simulink model "control_pmsm_multiple_wrapped"  (R2024b)
settings: Solver=FixedStepAuto  StartTime=0.0  StopTime=1  RelTol=1e-3  EnableMultiTasking=on
undefined symbols (not defined in the file): ControlModes, EstimationVelocityModes, InitConfParams, SupervisorEvents
settings Model: DataDictionary=amcfoc.sldd  Creator=upattacini  LastModifiedBy=mfussi
settings SolverCC: AllowMultiTaskInputOutput=on  AutoInsertRateTranBlk=on  InsertRTBMode=Never (minimum delay)  EnableFixedStepZeroCrossing=on
settings DataIOCC: SaveOutput=off  SignalLogging=off  DSMLogging=off  SaveTime=off
settings OptimizationCC: UseDivisionForNetSlopeComputation=on  SimCompilerOptimization=on
settings DebuggingCC: ParameterPrecisionLossMsg=none  UnconnectedInputMsg=warning  UnconnectedOutputMsg=warning  UnconnectedLineMsg=warning  BusObjectLabelMismatch=none
settings ModelReferenceCC: EnableRefExpFcnMdlSchedulingChecks=on  ModelReferenceMinAlgLoopOccurrences=on
settings SFSimCC: SimHardwareAcceleration=native
settings RTWCC: Toolchain=MinGW64 | gmake (64-bit Windows)  BuildConfiguration=Faster Runs  GPUComputeCapability=3.5  DLArmComputeVersion=19.05
settings GRTTargetCC: CodeInterfacePackaging=Reusable function  GenerateAllocFcn=on

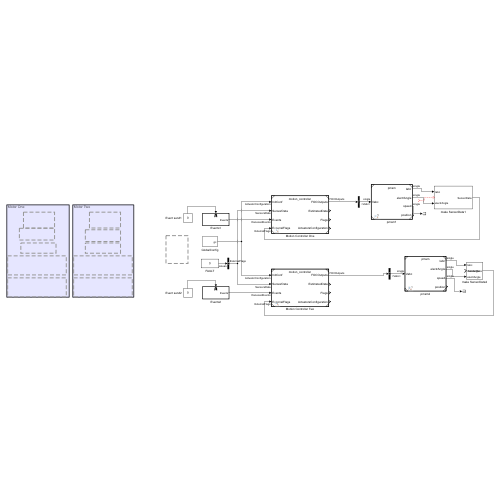
[thumbnail: Simulink's stored preview of the top-level diagram]
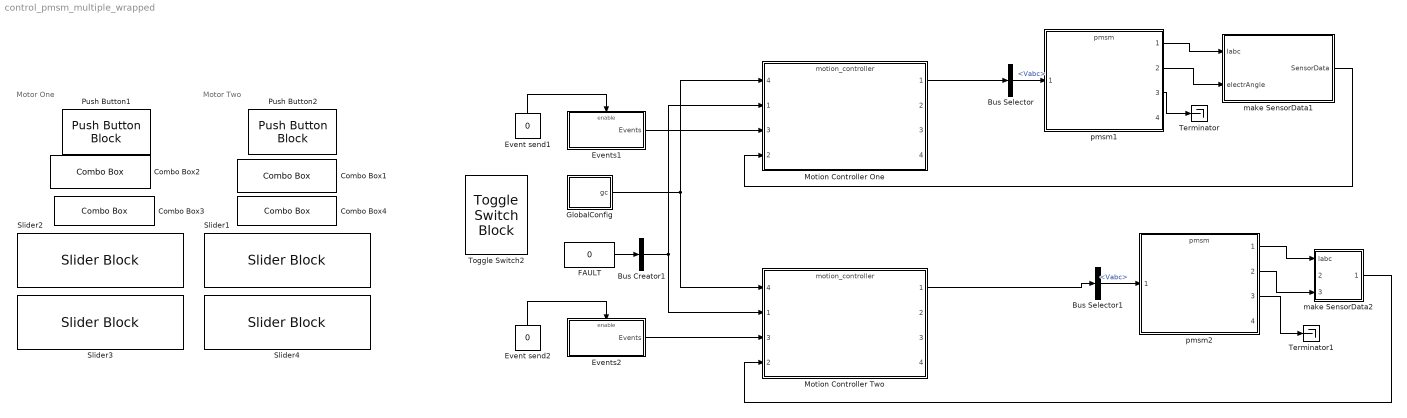
== system control_pmsm_multiple_wrapped ==
  note: Motor One
  note: Motor Two
  Bus Creator1 : BusCreator  Inputs=1  OutDataTypeStr=Bus: ExternalFlags  NonVirtualBus=on
      settings: InheritFromInputs=off
  Bus Selector : BusSelector  OutputSignals=Vabc
  Bus Selector1 : BusSelector  OutputSignals=Vabc
  Combo Box1 : ComboBox  SelectedLabel=None  UseEnumeratedDataType=on  EnumeratedDataType=SupervisorEvents
      settings: Values={{'None', 'SetLimit', 'SetControlMode', 'SetMotorConfig', 'SetPid', 'SetTarget'}, [0 1 2 5 3 4]}
  Combo Box2 : ComboBox  SelectedLabel=None  UseEnumeratedDataType=on  EnumeratedDataType=SupervisorEvents
      settings: Values={{'None', 'SetLimit', 'SetControlMode', 'SetMotorConfig', 'SetPid', 'SetTarget'}, [0 1 2 5 3 4]}
  Combo Box3 : ComboBox  SelectedLabel=Current  UseEnumeratedDataType=on  EnumeratedDataType=ControlModes
      settings: Values={{'NotConfigured', 'Idle', 'Position', 'PositionDirect', 'Current', 'Velocity', 'Voltage', 'Torque', 'HwFaultCM'}, [0 1 2 3 4 5 6 7 8]}
  Combo Box4 : ComboBox  SelectedLabel=Current  UseEnumeratedDataType=on  EnumeratedDataType=ControlModes
      settings: Values={{'NotConfigured', 'Idle', 'Position', 'PositionDirect', 'Current', 'Velocity', 'Voltage', 'Torque', 'HwFaultCM'}, [0 1 2 3 4 5 6 7 8]}
  Event send1 : Constant  Value=0
  Event send2 : Constant  Value=0
  Events1 : Subsystem
  Events2 : Subsystem
  FAULT : Constant  Value=0  OutDataTypeStr=Inherit: Inherit via back propagation
  GlobalConfig : Subsystem
  Motion Controller One : ModelReference  ModelNameDialog=motion_controller.slx  SimulationMode=Normal  ModelReferenceVersion=4.0
      settings: PortSchema="{\"entries\":[{\"content\":{\"sides\":[{\"content\":{\"connectorIds\":[\"In4\",\"In1\",\"In3\",\"In2\"]},\"type\":\"ConnectorPlacement.EquallySpacedRectSide\",\"uuid\":\"9501764e-0215-4e66-aa8b-5739ba26e582\"},{\"content\":{\"connectorIds\":[\"Out1\",\"Out2\",\"Out3\",\"Out4\"],\"side\":\"RIGHT\"},\"type\":\"ConnectorPlacement.EquallySpacedRectSide\",\"uuid\":\"34be47de-e9bc-43ca-97ac-58a43ba9eb9a\"},{\"content\":{\"side\":\"TOP\"},\"type\":\"ConnectorPlacement.EquallySpacedRectSide\",\"uuid\":\"71d421f6-ab26-4482-875c-bb9e44468ca7\"}]},\"type\":\"ConnectorPlacement.EquallySpacedConnector\",\"uuid\":\"be89792d-26da-4e9c-8783-03826ec72805\"}],\"packageUris\":[\"http://schema.mathworks.com/mf0/Connector/R2020b\"],\"version\":\"1.0\"}"
  Motion Controller Two : ModelReference  ModelNameDialog=motion_controller.slx  SimulationMode=Normal  ModelReferenceVersion=4.0
      settings: PortSchema="{\"entries\":[{\"content\":{\"sides\":[{\"content\":{\"connectorIds\":[\"In4\",\"In1\",\"In3\",\"In2\"]},\"type\":\"ConnectorPlacement.EquallySpacedRectSide\",\"uuid\":\"9501764e-0215-4e66-aa8b-5739ba26e582\"},{\"content\":{\"connectorIds\":[\"Out1\",\"Out2\",\"Out3\",\"Out4\"],\"side\":\"RIGHT\"},\"type\":\"ConnectorPlacement.EquallySpacedRectSide\",\"uuid\":\"34be47de-e9bc-43ca-97ac-58a43ba9eb9a\"},{\"content\":{\"side\":\"TOP\"},\"type\":\"ConnectorPlacement.EquallySpacedRectSide\",\"uuid\":\"71d421f6-ab26-4482-875c-bb9e44468ca7\"}]},\"type\":\"ConnectorPlacement.EquallySpacedConnector\",\"uuid\":\"be89792d-26da-4e9c-8783-03826ec72805\"}],\"packageUris\":[\"http://schema.mathworks.com/mf0/Connector/R2020b\"],\"version\":\"1.0\"}"
  Push Button1 : PushButtonBlock  LabelPosition=Top  OffValue=0.000000
  Push Button2 : PushButtonBlock  LabelPosition=Top  OffValue=0.000000
  Slider1 : SliderBlock  ScaleMax=1
  Slider2 : SliderBlock  ScaleMax=1
  Slider3 : SliderBlock  ScaleMax=0.36
  Slider4 : SliderBlock  ScaleMax=0.36
  Terminator : Terminator
  Terminator1 : Terminator
  Toggle Switch2 : ToggleSwitchBlock
      settings: Values={{'Off', 'On'}, [0 1]}
  make SensorData1 : Subsystem
  make SensorData2 : Subsystem
  pmsm1 : ModelReference  ModelNameDialog=pmsm.slx  SimulationMode=Normal  ModelReferenceVersion=9.5
  pmsm2 : ModelReference  ModelNameDialog=pmsm.slx  SimulationMode=Normal  ModelReferenceVersion=9.5
  wires:
  Event send1/1 -> Events1/Enable
  FAULT/1 -> Bus Creator1/1
  pmsm1/1 -> make SensorData1/1(Iabc)
  ? -> ?
  pmsm1/2 -> make SensorData1/2(electrAngle)
  pmsm2/1 -> make SensorData2/1(Iabc)
  pmsm2/2 -> make SensorData2/3(electrAngle)
  pmsm1/3 -> Terminator/1
  pmsm2/3 -> Terminator1/1
  Event send2/1 -> Events2/Enable
  Motion Controller One/1 -> Bus Selector/1
  Bus Selector/1 -> pmsm1/1  "<Vabc>"
  Motion Controller Two/1 -> Bus Selector1/1
  Bus Selector1/1 -> pmsm2/1  "<Vabc>"
  GlobalConfig/1(gc) -> Motion Controller One/4, Motion Controller Two/4
  Bus Creator1/1 -> Motion Controller One/1, Motion Controller Two/1
  Events1/1(Events) -> Motion Controller One/3
  make SensorData2/1(SensorData) -> Motion Controller Two/2
  Events2/1(Events) -> Motion Controller Two/3
  make SensorData1/1(SensorData) -> Motion Controller One/2

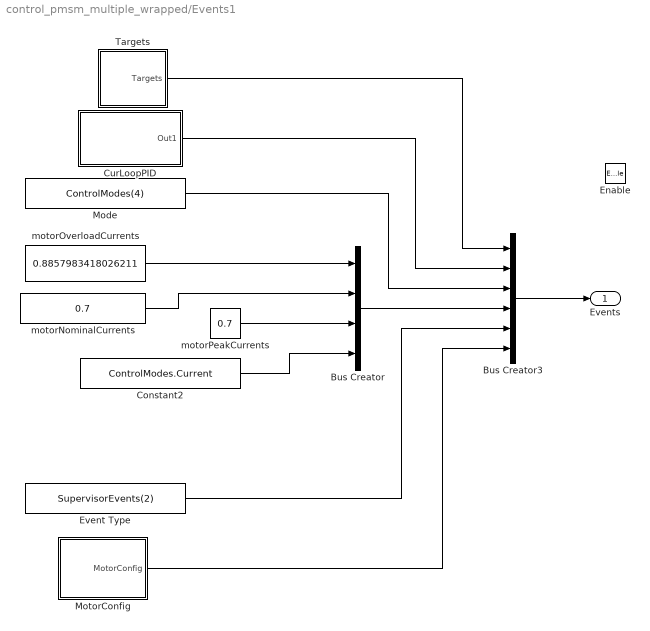
== system control_pmsm_multiple_wrapped/Events1 ==
  Enable : EnablePort
  Bus Creator : BusCreator  Inputs=4  OutDataTypeStr=Bus: SupervisorInputLimits
  Bus Creator3 : BusCreator  Inputs=6  OutDataTypeStr=Bus: SupervisorReceivedEvents  NonVirtualBus=on
      settings: InheritFromInputs=off
  Constant2 : Constant  Value=ControlModes.Current  OutDataTypeStr=Enum: ControlModes
  CurLoopPID : Subsystem  mask{OutMax=0, OutMin=0, P=2, I=500, D=0, N=10, I0=0, D0=0, shift_factor=0}
      mask prompts: shift_factor "Shift Factor"
  Event Type : Constant  Value=SupervisorEvents(2)  OutDataTypeStr=Enum: SupervisorEvents
  Mode : Constant  Value=ControlModes(4)  OutDataTypeStr=Enum: ControlModes
  MotorConfig : Subsystem  mask{has_hall_sens=InitConfParams(1).motor.has_hall_sens, has_quadrature_encoder=InitConfParams(1).motor.has_quadrature_encoder, has_speed_quadrature_encoder=InitConfParams(1).motor.has_speed_quadrature_encoder, has_torque_sens=InitConfParams(1).motor.has_torque_sens, use_index=InitConfParams(1).motor.use_index, enable_verbosity=InitConfParams(1).motor.enable_verbosity, rotor_encoder_resolution=InitConfParams(1).motor.rotor_encoder_resolution, rotor_index_offset=InitConfParams(1).motor.rotor_index_offset, encoder_tolerance=InitConfParams(1).motor.encoder_tolerance, pole_pairs=InitConfParams(1).motor.pole_pairs, reduction=100, Kbemf=InitConfParams(1).motor.Kbemf, Rphase=InitConfParams(1).motor.Rphase, Imin=InitConfParams(1).motor.Imin, Imax=InitConfParams(1).motor.Imax, Vcc=InitConfParams(1).motor.Vcc, Vmax=InitConfParams(1).motor.Vmax, R=InitConfParams(1).motor.resistance, L=InitConfParams(1).motor.inductance, Rt=InitConfParams(1).motor.thermal_resistance, tau=InitConfParams(1).motor.thermal_time_constant}
      mask prompts: R "Motor Resistance"; L "Motor Inductance"; Rt "Thermal Resistance"; tau "Thermal Time Constant"
  Targets : Subsystem
  motorNominalCurrents : Constant  Value=0.7  OutDataTypeStr=single
  motorOverloadCurrents : Constant  Value=0.8857983418026211  OutDataTypeStr=single
  motorPeakCurrents : Constant  Value=0.7  OutDataTypeStr=single
  Events : Outport
  wires:
  Bus Creator/1 -> Bus Creator3/4
  MotorConfig/1(MotorConfig) -> Bus Creator3/6
  Mode/1 -> Bus Creator3/3
  Targets/1(Targets) -> Bus Creator3/1
  Event Type/1 -> Bus Creator3/5
  CurLoopPID/1(Out1) -> Bus Creator3/2
  motorPeakCurrents/1 -> Bus Creator/3
  Constant2/1 -> Bus Creator/4
  motorOverloadCurrents/1 -> Bus Creator/1
  motorNominalCurrents/1 -> Bus Creator/2
  Bus Creator3/1 -> Events/1

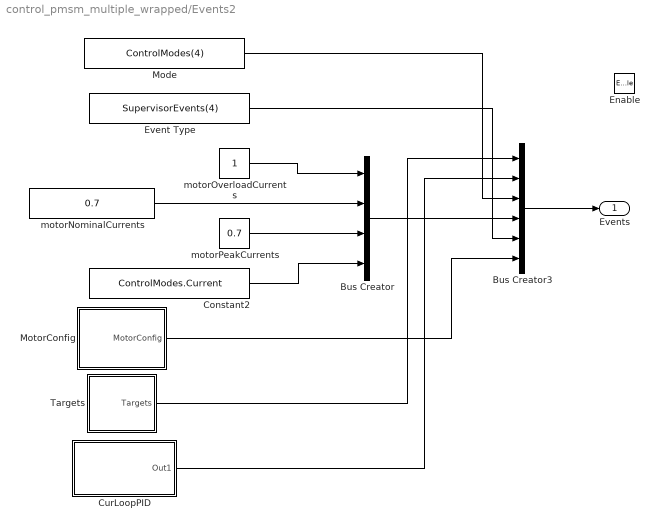
== system control_pmsm_multiple_wrapped/Events2 ==
  Enable : EnablePort
  Bus Creator : BusCreator  Inputs=4  OutDataTypeStr=Bus: SupervisorInputLimits
  Bus Creator3 : BusCreator  Inputs=6  OutDataTypeStr=Bus: SupervisorReceivedEvents  NonVirtualBus=on
      settings: InheritFromInputs=off
  Constant2 : Constant  Value=ControlModes.Current  OutDataTypeStr=Enum: ControlModes
  CurLoopPID : Subsystem  mask{OutMax=0, OutMin=0, P=2, I=500, D=0, N=10, I0=0, D0=0, shift_factor=0}
      mask prompts: shift_factor "Shift Factor"
  Event Type : Constant  Value=SupervisorEvents(4)  OutDataTypeStr=Enum: SupervisorEvents
  Mode : Constant  Value=ControlModes(4)  OutDataTypeStr=Enum: ControlModes
  MotorConfig : Subsystem  mask{has_hall_sens=InitConfParams(2).motor.has_hall_sens, has_quadrature_encoder=InitConfParams(2).motor.has_quadrature_encoder, has_speed_quadrature_encoder=InitConfParams(2).motor.has_speed_quadrature_encoder, has_torque_sens=InitConfParams(2).motor.has_torque_sens, use_index=InitConfParams(2).motor.use_index, enable_verbosity=InitConfParams(2).motor.enable_verbosity, rotor_encoder_resolution=InitConfParams(2).motor.rotor_encoder_resolution, rotor_index_offset=InitConfParams(2).motor.rotor_index_offset, encoder_tolerance=InitConfParams(2).motor.encoder_tolerance, pole_pairs=InitConfParams(2).motor.pole_pairs, reduction=100, Kbemf=InitConfParams(2).motor.Kbemf, Rphase=InitConfParams(2).motor.Rphase, Imin=InitConfParams(2).motor.Imin, Imax=InitConfParams(2).motor.Imax, Vcc=InitConfParams(2).motor.Vcc, Vmax=InitConfParams(2).motor.Vmax, R=InitConfParams(2).motor.resistance, L=InitConfParams(2).motor.inductance, Rt=InitConfParams(2).motor.thermal_resistance, tau=InitConfParams(2).motor.thermal_time_constant}
      mask prompts: R "Motor Resistance"; L "Motor Inductance"; Rt "Thermal Resistance"; tau "Thermal Time Constant"
  Targets : Subsystem
  motorNominalCurrents : Constant  Value=0.7  OutDataTypeStr=single
  motorOverloadCurrents : Constant  OutDataTypeStr=single
  motorPeakCurrents : Constant  Value=0.7  OutDataTypeStr=single
  Events : Outport
  wires:
  Bus Creator/1 -> Bus Creator3/4
  MotorConfig/1(MotorConfig) -> Bus Creator3/6
  Mode/1 -> Bus Creator3/3
  Targets/1(Targets) -> Bus Creator3/1
  Event Type/1 -> Bus Creator3/5
  CurLoopPID/1(Out1) -> Bus Creator3/2
  motorPeakCurrents/1 -> Bus Creator/3
  Constant2/1 -> Bus Creator/4
  motorOverloadCurrents/1 -> Bus Creator/1
  motorNominalCurrents/1 -> Bus Creator/2
  Bus Creator3/1 -> Events/1

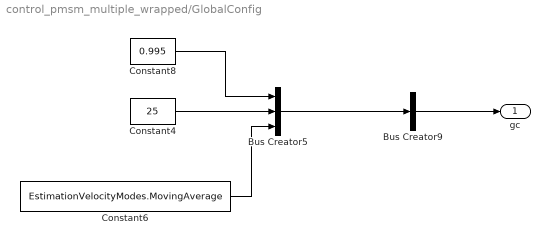
== system control_pmsm_multiple_wrapped/GlobalConfig ==
  Bus Creator5 : BusCreator  Inputs=3  OutDataTypeStr=Bus: EstimationConfiguration  NonVirtualBus=on
      settings: InheritFromInputs=off
  Bus Creator9 : BusCreator  Inputs=1  OutDataTypeStr=Bus: GlobalConfiguration  NonVirtualBus=on
      settings: InheritFromInputs=off
  Constant4 : Constant  Value=25  OutDataTypeStr=single
  Constant6 : Constant  Value=EstimationVelocityModes.MovingAverage  OutDataTypeStr=Enum: EstimationVelocityModes
  Constant8 : Constant  Value=0.995  OutDataTypeStr=single
  gc : Outport
  wires:
  Bus Creator9/1 -> gc/1
  Constant8/1 -> Bus Creator5/1
  Bus Creator5/1 -> Bus Creator9/1
  Constant4/1 -> Bus Creator5/2
  Constant6/1 -> Bus Creator5/3

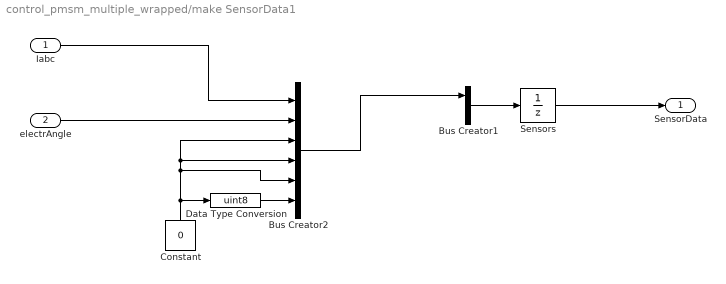
== system control_pmsm_multiple_wrapped/make SensorData1 ==
  Iabc : Inport
  electrAngle : Inport  Port=2
  Bus Creator1 : BusCreator  Inputs=2  OutDataTypeStr=Bus: SensorsData  NonVirtualBus=on
      settings: InheritFromInputs=off
  Bus Creator2 : BusCreator  Inputs=6  OutDataTypeStr=Bus: MotorSensors  NonVirtualBus=on
      settings: InheritFromInputs=off
  Constant : Constant  Value=0  OutDataTypeStr=single
  Data Type Conversion : DataTypeConversion  OutDataTypeStr=uint8  SaturateOnIntegerOverflow=off  RndMeth=Floor
  Sensors : UnitDelay  SampleTime=-1  HasFrameUpgradeWarning=on
  SensorData : Outport
  wires:
  Sensors/1 -> SensorData/1
  Constant/1 -> Bus Creator2/5, Bus Creator2/4, Bus Creator2/3, Data Type Conversion/1
  Iabc/1 -> Bus Creator2/1
  Bus Creator1/1 -> Sensors/1
  electrAngle/1 -> Bus Creator2/2
  Bus Creator2/1 -> Bus Creator1/1
  Data Type Conversion/1 -> Bus Creator2/6

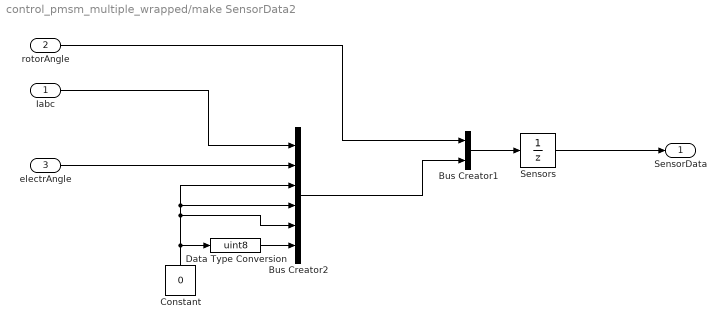
== system control_pmsm_multiple_wrapped/make SensorData2 ==
  Iabc : Inport
  rotorAngle : Inport  Port=2
  electrAngle : Inport  Port=3
  Bus Creator1 : BusCreator  Inputs=2  OutDataTypeStr=Bus: SensorsData  NonVirtualBus=on
      settings: InheritFromInputs=off
  Bus Creator2 : BusCreator  Inputs=6  OutDataTypeStr=Bus: MotorSensors  NonVirtualBus=on
      settings: InheritFromInputs=off
  Constant : Constant  Value=0  OutDataTypeStr=single
  Data Type Conversion : DataTypeConversion  OutDataTypeStr=uint8  SaturateOnIntegerOverflow=off  RndMeth=Floor
  Sensors : UnitDelay  SampleTime=-1  HasFrameUpgradeWarning=on
  SensorData : Outport
  wires:
  Sensors/1 -> SensorData/1
  Constant/1 -> Bus Creator2/5, Bus Creator2/4, Bus Creator2/3, Data Type Conversion/1
  Iabc/1 -> Bus Creator2/1
  rotorAngle/1 -> Bus Creator1/1
  Bus Creator1/1 -> Sensors/1
  electrAngle/1 -> Bus Creator2/2
  Bus Creator2/1 -> Bus Creator1/2
  Data Type Conversion/1 -> Bus Creator2/6

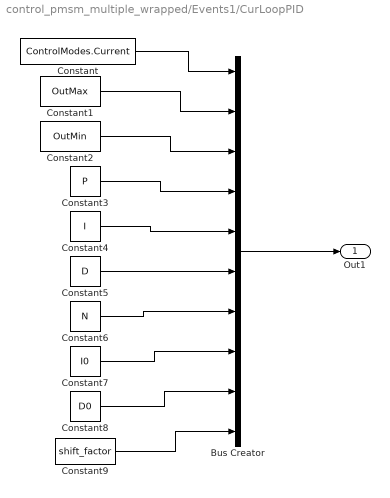
== system control_pmsm_multiple_wrapped/Events1/CurLoopPID ==
  Bus Creator : BusCreator  Inputs=10  OutDataTypeStr=Bus: PID
  Constant : Constant  Value=ControlModes.Current
  Constant1 : Constant  Value=OutMax  OutDataTypeStr=single
  Constant2 : Constant  Value=OutMin  OutDataTypeStr=single
  Constant3 : Constant  Value=P  OutDataTypeStr=single
  Constant4 : Constant  Value=I  OutDataTypeStr=single
  Constant5 : Constant  Value=D  OutDataTypeStr=single
  Constant6 : Constant  Value=N  OutDataTypeStr=single
  Constant7 : Constant  Value=I0  OutDataTypeStr=single
  Constant8 : Constant  Value=D0  OutDataTypeStr=single
  Constant9 : Constant  Value=shift_factor  OutDataTypeStr=uint8
  Out1 : Outport  OutDataTypeStr=Bus: PID
  wires:
  Bus Creator/1 -> Out1/1
  Constant8/1 -> Bus Creator/9
  Constant3/1 -> Bus Creator/4
  Constant5/1 -> Bus Creator/6
  Constant1/1 -> Bus Creator/2
  Constant7/1 -> Bus Creator/8
  Constant2/1 -> Bus Creator/3
  Constant9/1 -> Bus Creator/10
  Constant4/1 -> Bus Creator/5
  Constant/1 -> Bus Creator/1
  Constant6/1 -> Bus Creator/7

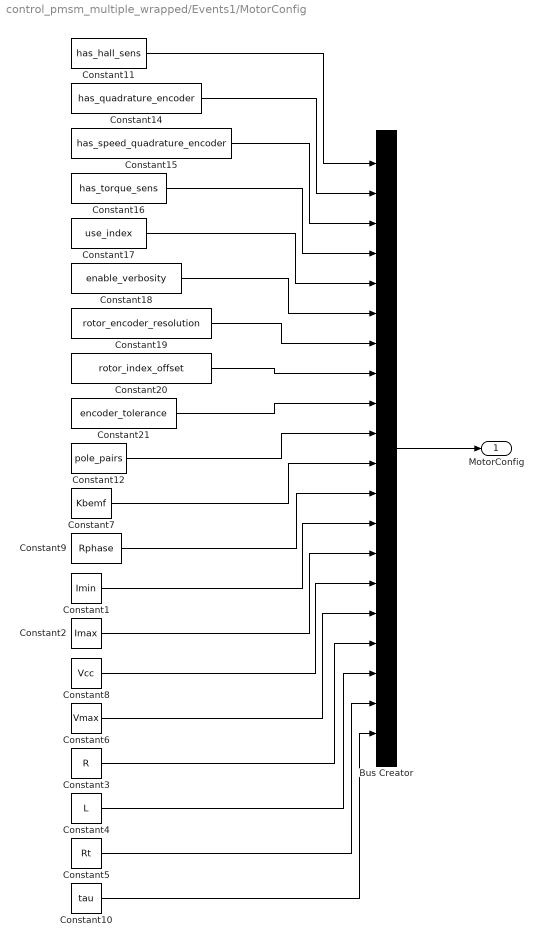
== system control_pmsm_multiple_wrapped/Events1/MotorConfig ==
  Bus Creator : BusCreator  Inputs=20  OutDataTypeStr=Bus: MotorConfiguration  NonVirtualBus=on
      settings: InheritFromInputs=off
  Constant1 : Constant  Value=Imin  OutDataTypeStr=single
  Constant10 : Constant  Value=tau  OutDataTypeStr=single
  Constant11 : Constant  Value=has_hall_sens  OutDataTypeStr=boolean
  Constant12 : Constant  Value=pole_pairs  OutDataTypeStr=uint8
  Constant14 : Constant  Value=has_quadrature_encoder  OutDataTypeStr=boolean
  Constant15 : Constant  Value=has_speed_quadrature_encoder  OutDataTypeStr=boolean
  Constant16 : Constant  Value=has_torque_sens  OutDataTypeStr=boolean
  Constant17 : Constant  Value=use_index  OutDataTypeStr=boolean
  Constant18 : Constant  Value=enable_verbosity  OutDataTypeStr=boolean
  Constant19 : Constant  Value=rotor_encoder_resolution  OutDataTypeStr=int16
  Constant2 : Constant  Value=Imax  OutDataTypeStr=single
  Constant20 : Constant  Value=rotor_index_offset  OutDataTypeStr=int16
  Constant21 : Constant  Value=encoder_tolerance  OutDataTypeStr=uint8
  Constant3 : Constant  Value=R  OutDataTypeStr=single
  Constant4 : Constant  Value=L  OutDataTypeStr=single
  Constant5 : Constant  Value=Rt  OutDataTypeStr=single
  Constant6 : Constant  Value=Vmax  OutDataTypeStr=single
  Constant7 : Constant  Value=Kbemf  OutDataTypeStr=single
  Constant8 : Constant  Value=Vcc  OutDataTypeStr=single
  Constant9 : Constant  Value=Rphase  OutDataTypeStr=single
  MotorConfig : Outport
  wires:
  Bus Creator/1 -> MotorConfig/1
  Constant20/1 -> Bus Creator/8
  Constant19/1 -> Bus Creator/7
  Constant21/1 -> Bus Creator/9
  Constant15/1 -> Bus Creator/3
  Constant18/1 -> Bus Creator/6
  Constant14/1 -> Bus Creator/2
  Constant16/1 -> Bus Creator/4
  Constant17/1 -> Bus Creator/5
  Constant12/1 -> Bus Creator/10
  Constant11/1 -> Bus Creator/1
  Constant7/1 -> Bus Creator/11
  Constant9/1 -> Bus Creator/12
  Constant1/1 -> Bus Creator/13
  Constant2/1 -> Bus Creator/14
  Constant8/1 -> Bus Creator/15
  Constant6/1 -> Bus Creator/16
  Constant3/1 -> Bus Creator/17
  Constant4/1 -> Bus Creator/18
  Constant5/1 -> Bus Creator/19
  Constant10/1 -> Bus Creator/20

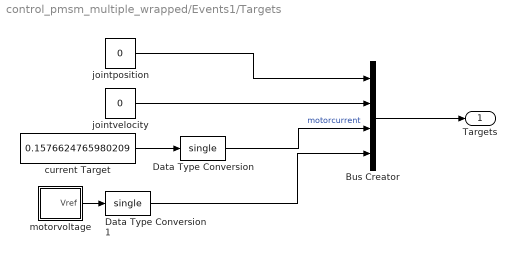
== system control_pmsm_multiple_wrapped/Events1/Targets ==
  Bus Creator : BusCreator  Inputs=4  OutDataTypeStr=Bus: Targets  NonVirtualBus=on
      settings: InheritFromInputs=off
  Data Type Conversion : DataTypeConversion  OutDataTypeStr=single  SaturateOnIntegerOverflow=off  RndMeth=Floor
  Data Type Conversion1 : DataTypeConversion  OutDataTypeStr=single  SaturateOnIntegerOverflow=off  RndMeth=Floor
  current Target : Constant  Value=0.1576624765980209
  jointposition : Constant  Value=0  OutDataTypeStr=single
  jointvelocity : Constant  Value=0  OutDataTypeStr=single
  motorvoltage : Subsystem
  Targets : Outport
  wires:
  Bus Creator/1 -> Targets/1
  jointposition/1 -> Bus Creator/1
  jointvelocity/1 -> Bus Creator/2
  Data Type Conversion1/1 -> Bus Creator/4
  Data Type Conversion/1 -> Bus Creator/3  "motorcurrent"
  motorvoltage/1(Vref) -> Data Type Conversion1/1
  current Target/1 -> Data Type Conversion/1

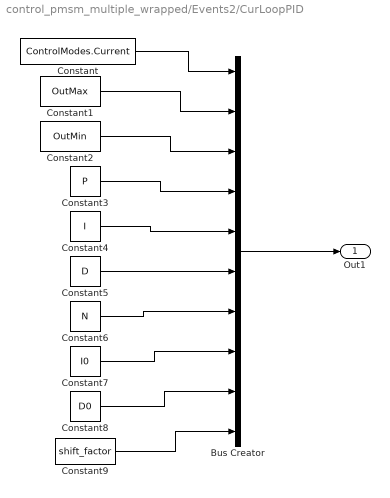
== system control_pmsm_multiple_wrapped/Events2/CurLoopPID ==
  Bus Creator : BusCreator  Inputs=10  OutDataTypeStr=Bus: PID
  Constant : Constant  Value=ControlModes.Current
  Constant1 : Constant  Value=OutMax  OutDataTypeStr=single
  Constant2 : Constant  Value=OutMin  OutDataTypeStr=single
  Constant3 : Constant  Value=P  OutDataTypeStr=single
  Constant4 : Constant  Value=I  OutDataTypeStr=single
  Constant5 : Constant  Value=D  OutDataTypeStr=single
  Constant6 : Constant  Value=N  OutDataTypeStr=single
  Constant7 : Constant  Value=I0  OutDataTypeStr=single
  Constant8 : Constant  Value=D0  OutDataTypeStr=single
  Constant9 : Constant  Value=shift_factor  OutDataTypeStr=uint8
  Out1 : Outport  OutDataTypeStr=Bus: PID
  wires:
  Bus Creator/1 -> Out1/1
  Constant8/1 -> Bus Creator/9
  Constant3/1 -> Bus Creator/4
  Constant5/1 -> Bus Creator/6
  Constant1/1 -> Bus Creator/2
  Constant7/1 -> Bus Creator/8
  Constant2/1 -> Bus Creator/3
  Constant9/1 -> Bus Creator/10
  Constant4/1 -> Bus Creator/5
  Constant/1 -> Bus Creator/1
  Constant6/1 -> Bus Creator/7

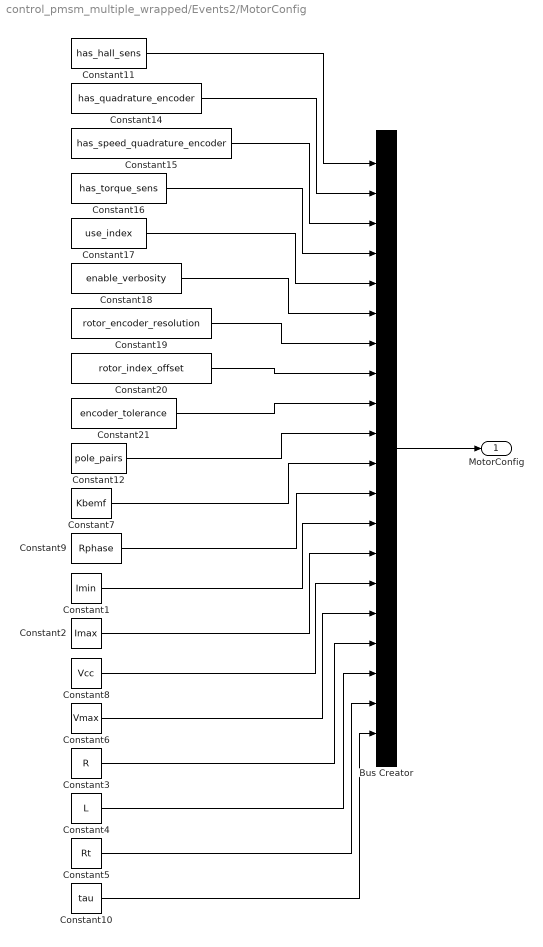
== system control_pmsm_multiple_wrapped/Events2/MotorConfig ==
  Bus Creator : BusCreator  Inputs=20  OutDataTypeStr=Bus: MotorConfiguration  NonVirtualBus=on
      settings: InheritFromInputs=off
  Constant1 : Constant  Value=Imin  OutDataTypeStr=single
  Constant10 : Constant  Value=tau  OutDataTypeStr=single
  Constant11 : Constant  Value=has_hall_sens  OutDataTypeStr=boolean
  Constant12 : Constant  Value=pole_pairs  OutDataTypeStr=uint8
  Constant14 : Constant  Value=has_quadrature_encoder  OutDataTypeStr=boolean
  Constant15 : Constant  Value=has_speed_quadrature_encoder  OutDataTypeStr=boolean
  Constant16 : Constant  Value=has_torque_sens  OutDataTypeStr=boolean
  Constant17 : Constant  Value=use_index  OutDataTypeStr=boolean
  Constant18 : Constant  Value=enable_verbosity  OutDataTypeStr=boolean
  Constant19 : Constant  Value=rotor_encoder_resolution  OutDataTypeStr=int16
  Constant2 : Constant  Value=Imax  OutDataTypeStr=single
  Constant20 : Constant  Value=rotor_index_offset  OutDataTypeStr=int16
  Constant21 : Constant  Value=encoder_tolerance  OutDataTypeStr=uint8
  Constant3 : Constant  Value=R  OutDataTypeStr=single
  Constant4 : Constant  Value=L  OutDataTypeStr=single
  Constant5 : Constant  Value=Rt  OutDataTypeStr=single
  Constant6 : Constant  Value=Vmax  OutDataTypeStr=single
  Constant7 : Constant  Value=Kbemf  OutDataTypeStr=single
  Constant8 : Constant  Value=Vcc  OutDataTypeStr=single
  Constant9 : Constant  Value=Rphase  OutDataTypeStr=single
  MotorConfig : Outport
  wires:
  Bus Creator/1 -> MotorConfig/1
  Constant20/1 -> Bus Creator/8
  Constant19/1 -> Bus Creator/7
  Constant21/1 -> Bus Creator/9
  Constant15/1 -> Bus Creator/3
  Constant18/1 -> Bus Creator/6
  Constant14/1 -> Bus Creator/2
  Constant16/1 -> Bus Creator/4
  Constant17/1 -> Bus Creator/5
  Constant12/1 -> Bus Creator/10
  Constant11/1 -> Bus Creator/1
  Constant7/1 -> Bus Creator/11
  Constant9/1 -> Bus Creator/12
  Constant1/1 -> Bus Creator/13
  Constant2/1 -> Bus Creator/14
  Constant8/1 -> Bus Creator/15
  Constant6/1 -> Bus Creator/16
  Constant3/1 -> Bus Creator/17
  Constant4/1 -> Bus Creator/18
  Constant5/1 -> Bus Creator/19
  Constant10/1 -> Bus Creator/20

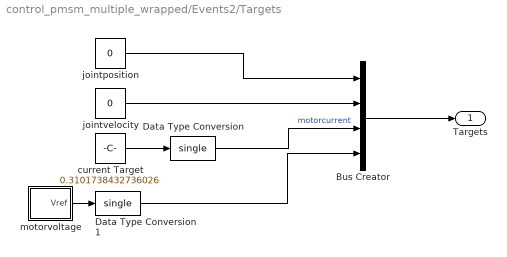
== system control_pmsm_multiple_wrapped/Events2/Targets ==
  Bus Creator : BusCreator  Inputs=4  OutDataTypeStr=Bus: Targets  NonVirtualBus=on
      settings: InheritFromInputs=off
  Data Type Conversion : DataTypeConversion  OutDataTypeStr=single  SaturateOnIntegerOverflow=off  RndMeth=Floor
  Data Type Conversion1 : DataTypeConversion  OutDataTypeStr=single  SaturateOnIntegerOverflow=off  RndMeth=Floor
  current Target : Constant  Value=0.3101738432736026  SampleTime=1e-3
  jointposition : Constant  Value=0  OutDataTypeStr=single  SampleTime=1e-3
  jointvelocity : Constant  Value=0  OutDataTypeStr=single  SampleTime=1e-3
  motorvoltage : Subsystem
  Targets : Outport
  wires:
  Bus Creator/1 -> Targets/1
  jointposition/1 -> Bus Creator/1
  jointvelocity/1 -> Bus Creator/2
  Data Type Conversion1/1 -> Bus Creator/4
  Data Type Conversion/1 -> Bus Creator/3  "motorcurrent"
  motorvoltage/1(Vref) -> Data Type Conversion1/1
  current Target/1 -> Data Type Conversion/1

== system control_pmsm_multiple_wrapped/Events1/Targets/motorvoltage ==
  Step : Step  Time=0.1  After=100
  Step1 : Step  Time=0.2  After=60
  Sum : Sum  Inputs=|+-
  Vref : Outport
  wires:
  Sum/1 -> Vref/1
  Step1/1 -> Sum/2
  Step/1 -> Sum/1

== system control_pmsm_multiple_wrapped/Events2/Targets/motorvoltage ==
  Step : Step  Time=0.1  After=100  SampleTime=1e-3
  Step1 : Step  Time=0.2  After=60  SampleTime=1e-3
  Sum : Sum  Inputs=|+-
  Vref : Outport
  wires:
  Sum/1 -> Vref/1
  Step1/1 -> Sum/2
  Step/1 -> Sum/1
